simulink model "sm_pump_triplex"  (R2025a)
settings: Solver=VariableStepAuto  StartTime=0.0  StopTime=1.5  RelTol=1e-3  EnableMultiTasking=on
undefined symbols (not defined in the file): pOut_Init_WKSP, smiData, TRP_Par, X, Y, Z
libraries: sm_lib x43, fl_lib x30, nesl_utility x11, simulink x10, SimscapeFluids_lib x3, sm_pump_triplex_lib x3, ee_lib x2, Multibody_Multiphysics_Lib x1
(part 3 of 3)

== system sm_pump_triplex/Pump/Crank/Crankpin 1 ==
  Shaft : sm_lib/Body Elements/Cylindrical Solid  CylinderRadius=shaft_rad  CylinderRadiusUnits=m  CylinderLength=shaft_len  CylinderLengthUnits=m  ExportEntireGeometry=off  InertiaType=CalculateFromGeometry  BasedOnType=Density  Density=crank_rho  DensityUnits=kg/m^3  Mass=1  MassUnits=kg  CenterOfMass=[0 0 0]  CenterOfMassUnits=m  MomentsOfInertia=[1 1 1]  MomentsOfInertiaUnits=kg*m^2  ProductsOfInertia=[1 1 1]  ProductsOfInertiaUnits=kg*m^2  GraphicType=FromGeometry  MarkerShape=Sphere  MarkerSize=10  GraphicVisPropType=SimpleVisualProperties  GraphicDiffuseColor=crank_clr  GraphicOpacity=crank_opc  GraphicSpecularColor=[0.5 0.5 0.5 1.0]  GraphicAmbientColor=[0.15 0.15 0.15 1.0]  GraphicEmissiveColor=[0.0 0.0 0.0 1.0]  GraphicShininess=75  DoExposeReferenceFrame=on  SerializedFrames=<Frames/>
  Transform S1 End : sm_lib/Frames and Transforms/Rigid Transform  RotationMethod=None  FollAlignAxisA=+X  BaseAlignAxisA=+Y  FollAlignAxisB=+Y  BaseAlignAxisB=+Z  RotationStandardAxis=+Z  RotationAngle=0.0  RotationAngleUnits=deg  RotationArbitraryAxis=[0 0 1]  RotationSequenceAxes=FollowerAxes  RotationSequence=XYX  RotationSequenceAngles=[0 0 0]  RotationSequenceAnglesUnits=deg  RotationMatrix=[1 0 0; 0 1 0; 0 0 1]  Quaternion=[1 0 0 0]  TranslationMethod=StandardAxis  TranslationCartesianOffset=[0 0 0]  TranslationCartesianOffsetUnits=m  TranslationStandardAxis=+Z  TranslationStandardOffset=shaft_len/2  TranslationStandardOffsetUnits=m  TranslationROffset=0  TranslationROffsetUnits=m  TranslationThetaOffset=0  TranslationThetaOffsetUnits=deg  TranslationZOffset=0  TranslationZOffsetUnits=m
  Transform S1 End1 : sm_lib/Frames and Transforms/Rigid Transform  RotationMethod=None  FollAlignAxisA=+X  BaseAlignAxisA=+Y  FollAlignAxisB=+Y  BaseAlignAxisB=+Z  RotationStandardAxis=+Z  RotationAngle=0.0  RotationAngleUnits=deg  RotationArbitraryAxis=[0 0 1]  RotationSequenceAxes=FollowerAxes  RotationSequence=XYX  RotationSequenceAngles=[0 0 0]  RotationSequenceAnglesUnits=deg  RotationMatrix=[1 0 0; 0 1 0; 0 0 1]  Quaternion=[1 0 0 0]  TranslationMethod=StandardAxis  TranslationCartesianOffset=[0 0 0]  TranslationCartesianOffsetUnits=m  TranslationStandardAxis=+Z  TranslationStandardOffset=shaft_len/2  TranslationStandardOffsetUnits=m  TranslationROffset=0  TranslationROffsetUnits=m  TranslationThetaOffset=0  TranslationThetaOffsetUnits=deg  TranslationZOffset=0  TranslationZOffsetUnits=m
  Transform Web 1 : sm_lib/Frames and Transforms/Rigid Transform  RotationMethod=None  FollAlignAxisA=+X  BaseAlignAxisA=+Y  FollAlignAxisB=+Y  BaseAlignAxisB=+Z  RotationStandardAxis=+Z  RotationAngle=0.0  RotationAngleUnits=deg  RotationArbitraryAxis=[0 0 1]  RotationSequenceAxes=FollowerAxes  RotationSequence=XYX  RotationSequenceAngles=[0 0 0]  RotationSequenceAnglesUnits=deg  RotationMatrix=[1 0 0; 0 1 0; 0 0 1]  Quaternion=[1 0 0 0]  TranslationMethod=Cylindrical  TranslationCartesianOffset=[0 0 0]  TranslationCartesianOffsetUnits=m  TranslationStandardAxis=+Z  TranslationStandardOffset=0  TranslationStandardOffsetUnits=m  TranslationROffset=shaft_pos  TranslationROffsetUnits=m  TranslationThetaOffset=120  TranslationThetaOffsetUnits=deg  TranslationZOffset=0  TranslationZOffsetUnits=m
  Transform Web 2 : sm_lib/Frames and Transforms/Rigid Transform  RotationMethod=None  FollAlignAxisA=+X  BaseAlignAxisA=+Y  FollAlignAxisB=+Y  BaseAlignAxisB=+Z  RotationStandardAxis=+Z  RotationAngle=0.0  RotationAngleUnits=deg  RotationArbitraryAxis=[0 0 1]  RotationSequenceAxes=FollowerAxes  RotationSequence=XYX  RotationSequenceAngles=[0 0 0]  RotationSequenceAnglesUnits=deg  RotationMatrix=[1 0 0; 0 1 0; 0 0 1]  Quaternion=[1 0 0 0]  TranslationMethod=Cylindrical  TranslationCartesianOffset=[0 0 0]  TranslationCartesianOffsetUnits=m  TranslationStandardAxis=+Z  TranslationStandardOffset=0  TranslationStandardOffsetUnits=m  TranslationROffset=shaft_pos  TranslationROffsetUnits=m  TranslationThetaOffset=-180+120  TranslationThetaOffsetUnits=deg  TranslationZOffset=0  TranslationZOffsetUnits=m
  W2 : PMIOPort  Side=Left
  P1 : PMIOPort  Port=2  Side=Right
  W1 : PMIOPort  Port=3  Side=Left
  connections:
  Transform Web 2/LConn1 -- Transform S1 End1/LConn1
  W2/RConn1 -- Transform Web 2/RConn1
  W1/RConn1 -- Transform Web 1/LConn1
  P1/RConn1 -- Shaft/RConn1 -- Transform S1 End/LConn1 -- Transform S1 End1/RConn1
  Transform Web 1/RConn1 -- Transform S1 End/RConn1

== system sm_pump_triplex/Pump/Crank/Crankpin 2 ==
  Shaft : sm_lib/Body Elements/Cylindrical Solid  CylinderRadius=shaft_rad  CylinderRadiusUnits=m  CylinderLength=shaft_len  CylinderLengthUnits=m  ExportEntireGeometry=off  InertiaType=CalculateFromGeometry  BasedOnType=Density  Density=crank_rho  DensityUnits=kg/m^3  Mass=1  MassUnits=kg  CenterOfMass=[0 0 0]  CenterOfMassUnits=m  MomentsOfInertia=[1 1 1]  MomentsOfInertiaUnits=kg*m^2  ProductsOfInertia=[1 1 1]  ProductsOfInertiaUnits=kg*m^2  GraphicType=FromGeometry  MarkerShape=Sphere  MarkerSize=10  GraphicVisPropType=SimpleVisualProperties  GraphicDiffuseColor=crank_clr  GraphicOpacity=crank_opc  GraphicSpecularColor=[0.5 0.5 0.5 1.0]  GraphicAmbientColor=[0.15 0.15 0.15 1.0]  GraphicEmissiveColor=[0.0 0.0 0.0 1.0]  GraphicShininess=75  DoExposeReferenceFrame=on  SerializedFrames=<Frames/>
  Transform S1 End : sm_lib/Frames and Transforms/Rigid Transform  RotationMethod=None  FollAlignAxisA=+X  BaseAlignAxisA=+Y  FollAlignAxisB=+Y  BaseAlignAxisB=+Z  RotationStandardAxis=+Z  RotationAngle=0.0  RotationAngleUnits=deg  RotationArbitraryAxis=[0 0 1]  RotationSequenceAxes=FollowerAxes  RotationSequence=XYX  RotationSequenceAngles=[0 0 0]  RotationSequenceAnglesUnits=deg  RotationMatrix=[1 0 0; 0 1 0; 0 0 1]  Quaternion=[1 0 0 0]  TranslationMethod=StandardAxis  TranslationCartesianOffset=[0 0 0]  TranslationCartesianOffsetUnits=m  TranslationStandardAxis=+Z  TranslationStandardOffset=shaft_len/2  TranslationStandardOffsetUnits=m  TranslationROffset=0  TranslationROffsetUnits=m  TranslationThetaOffset=0  TranslationThetaOffsetUnits=deg  TranslationZOffset=0  TranslationZOffsetUnits=m
  Transform S1 End1 : sm_lib/Frames and Transforms/Rigid Transform  RotationMethod=None  FollAlignAxisA=+X  BaseAlignAxisA=+Y  FollAlignAxisB=+Y  BaseAlignAxisB=+Z  RotationStandardAxis=+Z  RotationAngle=0.0  RotationAngleUnits=deg  RotationArbitraryAxis=[0 0 1]  RotationSequenceAxes=FollowerAxes  RotationSequence=XYX  RotationSequenceAngles=[0 0 0]  RotationSequenceAnglesUnits=deg  RotationMatrix=[1 0 0; 0 1 0; 0 0 1]  Quaternion=[1 0 0 0]  TranslationMethod=StandardAxis  TranslationCartesianOffset=[0 0 0]  TranslationCartesianOffsetUnits=m  TranslationStandardAxis=+Z  TranslationStandardOffset=shaft_len/2  TranslationStandardOffsetUnits=m  TranslationROffset=0  TranslationROffsetUnits=m  TranslationThetaOffset=0  TranslationThetaOffsetUnits=deg  TranslationZOffset=0  TranslationZOffsetUnits=m
  Transform Web 1 : sm_lib/Frames and Transforms/Rigid Transform  RotationMethod=None  FollAlignAxisA=+X  BaseAlignAxisA=+Y  FollAlignAxisB=+Y  BaseAlignAxisB=+Z  RotationStandardAxis=+Z  RotationAngle=0.0  RotationAngleUnits=deg  RotationArbitraryAxis=[0 0 1]  RotationSequenceAxes=FollowerAxes  RotationSequence=XYX  RotationSequenceAngles=[0 0 0]  RotationSequenceAnglesUnits=deg  RotationMatrix=[1 0 0; 0 1 0; 0 0 1]  Quaternion=[1 0 0 0]  TranslationMethod=Cylindrical  TranslationCartesianOffset=[0 0 0]  TranslationCartesianOffsetUnits=m  TranslationStandardAxis=+Z  TranslationStandardOffset=0  TranslationStandardOffsetUnits=m  TranslationROffset=shaft_pos  TranslationROffsetUnits=m  TranslationThetaOffset=0  TranslationThetaOffsetUnits=deg  TranslationZOffset=0  TranslationZOffsetUnits=m
  Transform Web 2 : sm_lib/Frames and Transforms/Rigid Transform  RotationMethod=None  FollAlignAxisA=+X  BaseAlignAxisA=+Y  FollAlignAxisB=+Y  BaseAlignAxisB=+Z  RotationStandardAxis=+Z  RotationAngle=0.0  RotationAngleUnits=deg  RotationArbitraryAxis=[0 0 1]  RotationSequenceAxes=FollowerAxes  RotationSequence=XYX  RotationSequenceAngles=[0 0 0]  RotationSequenceAnglesUnits=deg  RotationMatrix=[1 0 0; 0 1 0; 0 0 1]  Quaternion=[1 0 0 0]  TranslationMethod=Cylindrical  TranslationCartesianOffset=[0 0 0]  TranslationCartesianOffsetUnits=m  TranslationStandardAxis=+Z  TranslationStandardOffset=0  TranslationStandardOffsetUnits=m  TranslationROffset=shaft_pos  TranslationROffsetUnits=m  TranslationThetaOffset=-180  TranslationThetaOffsetUnits=deg  TranslationZOffset=0  TranslationZOffsetUnits=m
  W2 : PMIOPort  Side=Left
  P1 : PMIOPort  Port=2  Side=Right
  W1 : PMIOPort  Port=3  Side=Left
  connections:
  Transform Web 1/RConn1 -- Transform S1 End/RConn1
  Transform S1 End1/RConn1 -- Transform S1 End/LConn1 -- Shaft/RConn1 -- P1/RConn1
  W1/RConn1 -- Transform Web 1/LConn1
  W2/RConn1 -- Transform Web 2/RConn1
  Transform Web 2/LConn1 -- Transform S1 End1/LConn1

== system sm_pump_triplex/Pump/Crank/Crankpin 3 ==
  Shaft : sm_lib/Body Elements/Cylindrical Solid  CylinderRadius=shaft_rad  CylinderRadiusUnits=m  CylinderLength=shaft_len  CylinderLengthUnits=m  ExportEntireGeometry=off  InertiaType=CalculateFromGeometry  BasedOnType=Density  Density=crank_rho  DensityUnits=kg/m^3  Mass=1  MassUnits=kg  CenterOfMass=[0 0 0]  CenterOfMassUnits=m  MomentsOfInertia=[1 1 1]  MomentsOfInertiaUnits=kg*m^2  ProductsOfInertia=[1 1 1]  ProductsOfInertiaUnits=kg*m^2  GraphicType=FromGeometry  MarkerShape=Sphere  MarkerSize=10  GraphicVisPropType=SimpleVisualProperties  GraphicDiffuseColor=crank_clr  GraphicOpacity=crank_opc  GraphicSpecularColor=[0.5 0.5 0.5 1.0]  GraphicAmbientColor=[0.15 0.15 0.15 1.0]  GraphicEmissiveColor=[0.0 0.0 0.0 1.0]  GraphicShininess=75  DoExposeReferenceFrame=on  SerializedFrames=<Frames/>
  Transform S1 End : sm_lib/Frames and Transforms/Rigid Transform  RotationMethod=None  FollAlignAxisA=+X  BaseAlignAxisA=+Y  FollAlignAxisB=+Y  BaseAlignAxisB=+Z  RotationStandardAxis=+Z  RotationAngle=0.0  RotationAngleUnits=deg  RotationArbitraryAxis=[0 0 1]  RotationSequenceAxes=FollowerAxes  RotationSequence=XYX  RotationSequenceAngles=[0 0 0]  RotationSequenceAnglesUnits=deg  RotationMatrix=[1 0 0; 0 1 0; 0 0 1]  Quaternion=[1 0 0 0]  TranslationMethod=StandardAxis  TranslationCartesianOffset=[0 0 0]  TranslationCartesianOffsetUnits=m  TranslationStandardAxis=+Z  TranslationStandardOffset=shaft_len/2  TranslationStandardOffsetUnits=m  TranslationROffset=0  TranslationROffsetUnits=m  TranslationThetaOffset=0  TranslationThetaOffsetUnits=deg  TranslationZOffset=0  TranslationZOffsetUnits=m
  Transform S1 End1 : sm_lib/Frames and Transforms/Rigid Transform  RotationMethod=None  FollAlignAxisA=+X  BaseAlignAxisA=+Y  FollAlignAxisB=+Y  BaseAlignAxisB=+Z  RotationStandardAxis=+Z  RotationAngle=0.0  RotationAngleUnits=deg  RotationArbitraryAxis=[0 0 1]  RotationSequenceAxes=FollowerAxes  RotationSequence=XYX  RotationSequenceAngles=[0 0 0]  RotationSequenceAnglesUnits=deg  RotationMatrix=[1 0 0; 0 1 0; 0 0 1]  Quaternion=[1 0 0 0]  TranslationMethod=StandardAxis  TranslationCartesianOffset=[0 0 0]  TranslationCartesianOffsetUnits=m  TranslationStandardAxis=+Z  TranslationStandardOffset=shaft_len/2  TranslationStandardOffsetUnits=m  TranslationROffset=0  TranslationROffsetUnits=m  TranslationThetaOffset=0  TranslationThetaOffsetUnits=deg  TranslationZOffset=0  TranslationZOffsetUnits=m
  Transform Web 1 : sm_lib/Frames and Transforms/Rigid Transform  RotationMethod=None  FollAlignAxisA=+X  BaseAlignAxisA=+Y  FollAlignAxisB=+Y  BaseAlignAxisB=+Z  RotationStandardAxis=+Z  RotationAngle=0.0  RotationAngleUnits=deg  RotationArbitraryAxis=[0 0 1]  RotationSequenceAxes=FollowerAxes  RotationSequence=XYX  RotationSequenceAngles=[0 0 0]  RotationSequenceAnglesUnits=deg  RotationMatrix=[1 0 0; 0 1 0; 0 0 1]  Quaternion=[1 0 0 0]  TranslationMethod=Cylindrical  TranslationCartesianOffset=[0 0 0]  TranslationCartesianOffsetUnits=m  TranslationStandardAxis=+Z  TranslationStandardOffset=0  TranslationStandardOffsetUnits=m  TranslationROffset=shaft_pos  TranslationROffsetUnits=m  TranslationThetaOffset=-120  TranslationThetaOffsetUnits=deg  TranslationZOffset=0  TranslationZOffsetUnits=m
  Transform Web 2 : sm_lib/Frames and Transforms/Rigid Transform  RotationMethod=None  FollAlignAxisA=+X  BaseAlignAxisA=+Y  FollAlignAxisB=+Y  BaseAlignAxisB=+Z  RotationStandardAxis=+Z  RotationAngle=0.0  RotationAngleUnits=deg  RotationArbitraryAxis=[0 0 1]  RotationSequenceAxes=FollowerAxes  RotationSequence=XYX  RotationSequenceAngles=[0 0 0]  RotationSequenceAnglesUnits=deg  RotationMatrix=[1 0 0; 0 1 0; 0 0 1]  Quaternion=[1 0 0 0]  TranslationMethod=Cylindrical  TranslationCartesianOffset=[0 0 0]  TranslationCartesianOffsetUnits=m  TranslationStandardAxis=+Z  TranslationStandardOffset=0  TranslationStandardOffsetUnits=m  TranslationROffset=shaft_pos  TranslationROffsetUnits=m  TranslationThetaOffset=-180-120  TranslationThetaOffsetUnits=deg  TranslationZOffset=0  TranslationZOffsetUnits=m
  W2 : PMIOPort  Side=Left
  P1 : PMIOPort  Port=2  Side=Right
  W1 : PMIOPort  Port=3  Side=Left
  connections:
  Transform Web 2/LConn1 -- Transform S1 End1/LConn1
  W2/RConn1 -- Transform Web 2/RConn1
  W1/RConn1 -- Transform Web 1/LConn1
  P1/RConn1 -- Shaft/RConn1 -- Transform S1 End/LConn1 -- Transform S1 End1/RConn1
  Transform Web 1/RConn1 -- Transform S1 End/RConn1

== system sm_pump_triplex/Pump/Housing/Bearing Fault Visual ==
  Bearing Fault Visual L : sm_lib/Body Elements/Cylindrical Solid  CylinderRadius=bearing_fault_vis_rad  CylinderRadiusUnits=m  CylinderLength=bearing_fault_vis_len  CylinderLengthUnits=m  ExportEntireGeometry=off  InertiaType=CalculateFromGeometry  BasedOnType=Density  Density=0.001  DensityUnits=kg/m^3  Mass=1  MassUnits=kg  CenterOfMass=[0 0 0]  CenterOfMassUnits=m  MomentsOfInertia=[1 1 1]  MomentsOfInertiaUnits=kg*m^2  ProductsOfInertia=[1 1 1]  ProductsOfInertiaUnits=kg*m^2  GraphicType=FromGeometry  MarkerShape=Sphere  MarkerSize=10  GraphicVisPropType=SimpleVisualProperties  GraphicDiffuseColor=bearing_fault_vis_clr  GraphicOpacity=bearing_fault_vis_opc  GraphicSpecularColor=[0.5 0.5 0.5 1.0]  GraphicAmbientColor=[0.15 0.15 0.15 1.0]  GraphicEmissiveColor=[0.0 0.0 0.0 1.0]  GraphicShininess=75  DoExposeReferenceFrame=on  SerializedFrames=<Frames/>
  Bearing Fault Visual R : sm_lib/Body Elements/Cylindrical Solid  CylinderRadius=bearing_fault_vis_rad  CylinderRadiusUnits=m  CylinderLength=bearing_fault_vis_len  CylinderLengthUnits=m  ExportEntireGeometry=off  InertiaType=CalculateFromGeometry  BasedOnType=Density  Density=0.001  DensityUnits=kg/m^3  Mass=1  MassUnits=kg  CenterOfMass=[0 0 0]  CenterOfMassUnits=m  MomentsOfInertia=[1 1 1]  MomentsOfInertiaUnits=kg*m^2  ProductsOfInertia=[1 1 1]  ProductsOfInertiaUnits=kg*m^2  GraphicType=FromGeometry  MarkerShape=Sphere  MarkerSize=10  GraphicVisPropType=SimpleVisualProperties  GraphicDiffuseColor=bearing_fault_vis_clr  GraphicOpacity=bearing_fault_vis_opc  GraphicSpecularColor=[0.5 0.5 0.5 1.0]  GraphicAmbientColor=[0.15 0.15 0.15 1.0]  GraphicEmissiveColor=[0.0 0.0 0.0 1.0]  GraphicShininess=75  DoExposeReferenceFrame=on  SerializedFrames=<Frames/>
  Transform Bearing Fault L : sm_lib/Frames and Transforms/Rigid Transform  RotationMethod=None  FollAlignAxisA=+X  BaseAlignAxisA=+Y  FollAlignAxisB=+Y  BaseAlignAxisB=+Z  RotationStandardAxis=+Z  RotationAngle=0.0  RotationAngleUnits=deg  RotationArbitraryAxis=[0 0 1]  RotationSequenceAxes=FollowerAxes  RotationSequence=XYX  RotationSequenceAngles=[0 0 0]  RotationSequenceAnglesUnits=deg  RotationMatrix=[1 0 0; 0 1 0; 0 0 1]  Quaternion=[1 0 0 0]  TranslationMethod=StandardAxis  TranslationCartesianOffset=[0 0 0]  TranslationCartesianOffsetUnits=m  TranslationStandardAxis=+Z  TranslationStandardOffset=bearing_sep/2  TranslationStandardOffsetUnits=m  TranslationROffset=0  TranslationROffsetUnits=m  TranslationThetaOffset=0  TranslationThetaOffsetUnits=deg  TranslationZOffset=0  TranslationZOffsetUnits=m
  Transform Bearing Fault R : sm_lib/Frames and Transforms/Rigid Transform  RotationMethod=None  FollAlignAxisA=+X  BaseAlignAxisA=+Y  FollAlignAxisB=+Y  BaseAlignAxisB=+Z  RotationStandardAxis=+Z  RotationAngle=0.0  RotationAngleUnits=deg  RotationArbitraryAxis=[0 0 1]  RotationSequenceAxes=FollowerAxes  RotationSequence=XYX  RotationSequenceAngles=[0 0 0]  RotationSequenceAnglesUnits=deg  RotationMatrix=[1 0 0; 0 1 0; 0 0 1]  Quaternion=[1 0 0 0]  TranslationMethod=StandardAxis  TranslationCartesianOffset=[0 0 0]  TranslationCartesianOffsetUnits=m  TranslationStandardAxis=-Z  TranslationStandardOffset=bearing_sep/2  TranslationStandardOffsetUnits=m  TranslationROffset=0  TranslationROffsetUnits=m  TranslationThetaOffset=0  TranslationThetaOffsetUnits=deg  TranslationZOffset=0  TranslationZOffsetUnits=m
  C : PMIOPort  Side=Left
  connections:
  Transform Bearing Fault L/LConn1 -- Transform Bearing Fault R/LConn1 -- C/RConn1
  Bearing Fault Visual R/RConn1 -- Transform Bearing Fault R/RConn1
  Bearing Fault Visual L/RConn1 -- Transform Bearing Fault L/RConn1

== system sm_pump_triplex/Pump/Housing/Shell ==
  Housing_1_RIGID : Subsystem
  Manifold_1_RIGID : Subsystem
  Transform : sm_lib/Frames and Transforms/Rigid Transform  RotationMethod=ArbitraryAxis  FollAlignAxisA=+X  BaseAlignAxisA=+Y  FollAlignAxisB=+Y  BaseAlignAxisB=+Z  RotationStandardAxis=+Z  RotationAngle=smiData.RigidTransform(9).angle  RotationAngleUnits=rad  RotationArbitraryAxis=smiData.RigidTransform(9).axis  RotationSequenceAxes=FollowerAxes  RotationSequence=XYX  RotationSequenceAngles=[0 0 0]  RotationSequenceAnglesUnits=deg  RotationMatrix=[1 0 0; 0 1 0; 0 0 1]  Quaternion=[1 0 0 0]  TranslationMethod=Cartesian  TranslationCartesianOffset=smiData.RigidTransform(9).translation  TranslationCartesianOffsetUnits=in  TranslationStandardAxis=+Z  TranslationStandardOffset=0  TranslationStandardOffsetUnits=in  TranslationROffset=0  TranslationROffsetUnits=m  TranslationThetaOffset=0  TranslationThetaOffsetUnits=deg  TranslationZOffset=0  TranslationZOffsetUnits=m
  Transform1 : sm_lib/Frames and Transforms/Rigid Transform  RotationMethod=ArbitraryAxis  FollAlignAxisA=+X  BaseAlignAxisA=+Y  FollAlignAxisB=+Y  BaseAlignAxisB=+Z  RotationStandardAxis=+Z  RotationAngle=smiData.RigidTransform(10).angle  RotationAngleUnits=rad  RotationArbitraryAxis=smiData.RigidTransform(10).axis  RotationSequenceAxes=FollowerAxes  RotationSequence=XYX  RotationSequenceAngles=[0 0 0]  RotationSequenceAnglesUnits=deg  RotationMatrix=[1 0 0; 0 1 0; 0 0 1]  Quaternion=[1 0 0 0]  TranslationMethod=Cartesian  TranslationCartesianOffset=smiData.RigidTransform(10).translation  TranslationCartesianOffsetUnits=in  TranslationStandardAxis=+Z  TranslationStandardOffset=0  TranslationStandardOffsetUnits=in  TranslationROffset=0  TranslationROffsetUnits=m  TranslationThetaOffset=0  TranslationThetaOffsetUnits=deg  TranslationZOffset=0  TranslationZOffsetUnits=m
  W : PMIOPort  Side=Left
  connections:
  Transform1/LConn1 -- W/RConn1 -- Transform/LConn1
  Manifold_1_RIGID/LConn1 -- Transform/RConn1
  Housing_1_RIGID/LConn1 -- Transform1/RConn1

== system sm_pump_triplex/Driver/Driver/Dyno/Sensing Speed ==
  w : Inport
  Measurement Noise : simulink/Sources/Band-Limited White Noise  Cov=TRP_Par.Sensors.w.Np  Ts=TRP_Par.Sensors.w.Ts  seed=[23345]
  Motor Gear Ratio : Gain  Gain=TRP_Par.Motor.Gear.ratio
  Speed with Noise : Scope  NumInputPorts=2
      settings: ActiveDisplayYMinimum=-126.98875  ActiveDisplayYMaximum=1142.56233
  Sum1 : Sum  Inputs=++|
  Zero-Order Hold : ZeroOrderHold  SampleTime=TRP_Par.Sensors.w.Ts
  wires:
  Measurement Noise/1 -> Sum1/1  "Noise"
  w/1 -> Motor Gear Ratio/1
  Sum1/1 -> Zero-Order Hold/1
  Zero-Order Hold/1 -> Speed with Noise/1
  Motor Gear Ratio/1 -> Sum1/2, Speed with Noise/2

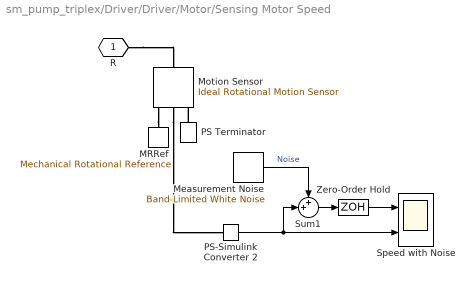
== system sm_pump_triplex/Driver/Driver/Motor/Sensing Motor Speed ==
  MRRef : fl_lib/Mechanical/Rotational Elements/Mechanical Rotational Reference
  Measurement Noise : simulink/Sources/Band-Limited White Noise  Cov=TRP_Par.Sensors.w.Np  Ts=TRP_Par.Sensors.w.Ts  seed=[23345]
  Motion Sensor : fl_lib/Mechanical/Mechanical Sensors/Ideal Rotational Motion Sensor  reference=foundation.enum.MeasurementReference.difference  acceleration_port=false  velocity_port=true  position_port=true  wrap_angle=simscape.enum.onoff.off  offset=0 rad
  PS Terminator : fl_lib/Physical Signals/Sinks/PS Terminator
  PS-Simulink Converter 2 : nesl_utility/PS-Simulink Converter  PhysicalDomain=network_engine_domain  SubClassName=ps_output  LeftPortType=input  RightPortType=output  PseudoPeriodic=off  Frequencies=[]  VectorFormat=1-D array  Unit=rpm  AffineConversion=off
  Speed with Noise : Scope  NumInputPorts=2
      settings: ActiveDisplayYMinimum=-126.98875  ActiveDisplayYMaximum=1142.56233
  Sum1 : Sum  Inputs=++|
  Zero-Order Hold : ZeroOrderHold  SampleTime=TRP_Par.Sensors.w.Ts
  R : PMIOPort  Side=Left
  wires:
  Measurement Noise/1 -> Sum1/1  "Noise"
  PS-Simulink Converter 2/1 -> Speed with Noise/2, Sum1/2
  Zero-Order Hold/1 -> Speed with Noise/1
  Sum1/1 -> Zero-Order Hold/1
  connections:
  PS Terminator/LConn1 -- Motion Sensor/RConn3
  R/RConn1 -- Motion Sensor/LConn1
  Motion Sensor/RConn1 -- MRRef/LConn1
  Motion Sensor/RConn2 -- PS-Simulink Converter 2/LConn1

== system sm_pump_triplex/Driver/Driver/Motor/Sensing Pump Speed ==
  MRRef : fl_lib/Mechanical/Rotational Elements/Mechanical Rotational Reference
  Motion Sensor : fl_lib/Mechanical/Mechanical Sensors/Ideal Rotational Motion Sensor  reference=foundation.enum.MeasurementReference.difference  acceleration_port=false  velocity_port=true  position_port=true  wrap_angle=simscape.enum.onoff.off  offset=0 rad
  PS-Simulink Converter 1 : nesl_utility/PS-Simulink Converter  PhysicalDomain=network_engine_domain  SubClassName=ps_output  LeftPortType=input  RightPortType=output  PseudoPeriodic=off  Frequencies=[]  VectorFormat=1-D array  Unit=deg  AffineConversion=off
  PS-Simulink Converter 2 : nesl_utility/PS-Simulink Converter  PhysicalDomain=network_engine_domain  SubClassName=ps_output  LeftPortType=input  RightPortType=output  PseudoPeriodic=off  Frequencies=[]  VectorFormat=1-D array  Unit=rpm  AffineConversion=off
  R : PMIOPort  Side=Left
  A : Outport  VectorParamsAs1DForOutWhenUnconnected=off
  rpm : Outport  Port=2  VectorParamsAs1DForOutWhenUnconnected=off
  wires:
  PS-Simulink Converter 1/1 -> A/1
  PS-Simulink Converter 2/1 -> rpm/1
  connections:
  Motion Sensor/RConn2 -- PS-Simulink Converter 2/LConn1
  Motion Sensor/RConn1 -- MRRef/LConn1
  R/RConn1 -- Motion Sensor/LConn1
  Motion Sensor/RConn3 -- PS-Simulink Converter 1/LConn1

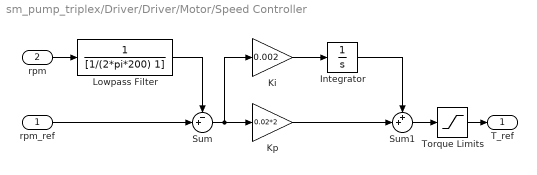
== system sm_pump_triplex/Driver/Driver/Motor/Speed Controller ==
  rpm_ref : Inport
  rpm : Inport  Port=2
  Integrator : Integrator  LimitOutput=on  UpperSaturationLimit=40  LowerSaturationLimit=-40
      settings: AttributesFormatString=Saturate: [%<LowerSaturationLimit>, %<UpperSaturationLimit>]
  Ki : Gain  Gain=0.002
  Kp : Gain  Gain=0.02*2
  Lowpass Filter : TransferFcn  Denominator=[1/(2*pi*200) 1]
  Sum : Sum  Inputs=-+|
  Sum1 : Sum  Inputs=++|
  Torque Limits : Saturate  UpperLimit=400  LowerLimit=-400
  T_ref : Outport  VectorParamsAs1DForOutWhenUnconnected=off
  wires:
  rpm_ref/1 -> Sum/2
  rpm/1 -> Lowpass Filter/1
  Sum1/1 -> Torque Limits/1
  Sum/1 -> Ki/1, Kp/1
  Ki/1 -> Integrator/1
  Kp/1 -> Sum1/2
  Integrator/1 -> Sum1/1
  Lowpass Filter/1 -> Sum/1
  Torque Limits/1 -> T_ref/1

== system sm_pump_triplex/Driver/Driver/Motor/Windings ==
  T_ref : Inport
  deg : Inport  Port=2
  Constant : Constant  Value=winding_fault_sw
  Constant1 : Constant
  Enable if rotor angle 0-240 Deg : Subsystem
  Product : Product
  Switch : Switch  Criteria=u2 > Threshold  Threshold=1.5  SaturateOnIntegerOverflow=off  InputSameDT=off
  Unit Delay : UnitDelay  SampleTime=0.001  HasFrameUpgradeWarning=on
  Trq : Outport  VectorParamsAs1DForOutWhenUnconnected=off
  wires:
  Product/1 -> Trq/1
  T_ref/1 -> Product/1
  Constant/1 -> Switch/2
  Constant1/1 -> Switch/3
  Switch/1 -> Product/2
  deg/1 -> Unit Delay/1
  Enable if rotor angle 0-240 Deg/1(En) -> Switch/1
  Unit Delay/1 -> Enable if rotor angle 0-240 Deg/1(Ang)

== system sm_pump_triplex/Pump/Housing/Shell/Housing_1_RIGID ==
  ReferenceFrame : sm_lib/Frames and Transforms/Reference Frame
  Solid : sm_lib/Body Elements/File Solid  ExtGeomFileName=Housing_Default_sldprt.STEP  UnitType=FromFile  ExtGeomFileUnits=m  StepReaderType=HEX  ExportConvexHullGeometry=off  InertiaType=Custom  BasedOnType=Density  Density=1000  DensityUnits=kg/m^3  Mass=smiData.Solid(4).mass  MassUnits=kg  CenterOfMass=smiData.Solid(4).CoM  CenterOfMassUnits=in  MomentsOfInertia=smiData.Solid(4).MoI  MomentsOfInertiaUnits=kg*in^2  ProductsOfInertia=smiData.Solid(4).PoI  ProductsOfInertiaUnits=kg*in^2  GraphicType=FromGeometry  MarkerShape=Sphere  MarkerSize=10  GraphicVisPropType=SimpleVisualProperties  GraphicDiffuseColor=housing_clr  GraphicOpacity=housing_opc  GraphicSpecularColor=[0.5 0.5 0.5 1.0]  GraphicAmbientColor=[0.15 0.15 0.15 1.0]  GraphicEmissiveColor=[0.0 0.0 0.0 1.0]  GraphicShininess=75  DoExposeReferenceFrame=on  SerializedFrames=<Frames/>
  F : PMIOPort  Side=Left
  connections:
  Solid/RConn1 -- ReferenceFrame/RConn1 -- F/RConn1

== system sm_pump_triplex/Pump/Housing/Shell/Manifold_1_RIGID ==
  ReferenceFrame : sm_lib/Frames and Transforms/Reference Frame
  Solid : sm_lib/Body Elements/File Solid  ExtGeomFileName=Manifold_Default_sldprt.STEP  UnitType=FromFile  ExtGeomFileUnits=m  StepReaderType=HEX  ExportConvexHullGeometry=off  InertiaType=Custom  BasedOnType=Density  Density=1000  DensityUnits=kg/m^3  Mass=smiData.Solid(3).mass  MassUnits=kg  CenterOfMass=smiData.Solid(3).CoM  CenterOfMassUnits=in  MomentsOfInertia=smiData.Solid(3).MoI  MomentsOfInertiaUnits=kg*in^2  ProductsOfInertia=smiData.Solid(3).PoI  ProductsOfInertiaUnits=kg*in^2  GraphicType=FromGeometry  MarkerShape=Sphere  MarkerSize=10  GraphicVisPropType=SimpleVisualProperties  GraphicDiffuseColor=manifold_clr  GraphicOpacity=manifold_opc  GraphicSpecularColor=[0.5 0.5 0.5 1.0]  GraphicAmbientColor=[0.15 0.15 0.15 1.0]  GraphicEmissiveColor=[0.0 0.0 0.0 1.0]  GraphicShininess=75  DoExposeReferenceFrame=on  SerializedFrames=<Frames/>
  F : PMIOPort  Side=Left
  connections:
  Solid/RConn1 -- ReferenceFrame/RConn1 -- F/RConn1

== system sm_pump_triplex/Driver/Driver/Motor/Windings/Enable if rotor angle 0-240 Deg ==
  Ang : Inport
  Constant2 : Constant  Value=360
  Interval Test : simulink/Logic and Bit Operations/Interval Test  IntervalClosedRight=on  uplimit=240  IntervalClosedLeft=on  lowlimit=0  OutDataTypeStr=uint8
      settings: AttributesFormatString=%<lowlimit><angle<%<uplimit>
  Math Function : Math  Operator=rem  SignedPower=on
  En : Outport  VectorParamsAs1DForOutWhenUnconnected=off
  wires:
  Constant2/1 -> Math Function/2
  Math Function/1 -> Interval Test/1
  Interval Test/1 -> En/1
  Ang/1 -> Math Function/1

== matlab function sm_pump_triplex/Diagnostics/Diagnostics/On/FFT and Classification ==
  data: pArray input; faultState output; enablePred input; cmdSpeed input; hmiVec output
function [faultState,hmiVec] = faultClassifier(pArray,enablePred,cmdSpeed)

% Initialize Predicted Machine State
faultState = int8(0);
hmiVec = [1 0 0 0];

% Sampling Parameters
Np = 1000;
Dt = 0.001;
numFreqPeaks = 5;

% Initialize Prediction Algorithm Input
predIn = NaN(1,2*numFreqPeaks+1);

pAvg = mean(pArray);

% Load Trained Machine Learning Algorithm
pumpPredict = loadLearnerForCoder('sm_pump_triplex_fault_detect_algo');

if enablePred
    
    % Compute FFT of Accumulated Data
    [freq,mag] = getFFTData(Np,pArray,Dt);
    
    % Normalize FFT Results
    freqFaultSpd = freq*60/(2*pi)/(cmdSpeed*3);

    % Detect FFT Peak Frequencies
    [pks,loc] = findpeaks(mag,'MinPeakProminence',0.5e-3);

    % Center FFT Peak Frequencies around Primary Machine Frequency
    normSpd = abs(freqFaultSpd(loc)-1);
    [sortFreq,sortIdx] = sort(normSpd);
    sortMag = pks(sortIdx);

    % Only Update Detected Peaks
    if length(sortMag) <= numFreqPeaks
        numFreq = length(sortMag);
    else
        numFreq = numFreqPeaks;
    end
    
    % Construct Input Array for Machine Learning Algorithm
    for i = 1:numFreq
        predIn(2*(i-1)+1) = sortFreq(i);
        predIn(2*i) = sortMag(i);
        predIn(i+1) = sortMag(i);
    end
    predIn(2*numFreqPeaks+1) = pAvg;
    
    % Predict Machine State using Classification Algorithm
    faultState = predict(pumpPredict,predIn);
    
    % Flag Machine Vector for HMI Indicators
    if faultState == 3 || faultState == 4 || faultState == 5
        hmiVec(2) = 1;  hmiVec(1) = 0;
    end
    if faultState == 1 || faultState == 2 || faultState == 4
        hmiVec(3) = 1;  hmiVec(1) = 0;
    end
    if faultState == 2 || faultState == 5 || faultState == 7
        hmiVec(4) = 1;  hmiVec(1) = 0;
    end
    
else
    % 
    faultState = int8(0);
    hmiVec = [0 0 0 0];
end
end

function [freq, mag] = getFFTData(np,yout,dt)
% Code to calculate frequency response data
%
% Copyright 2017 The MathWorks, Inc.

% % Compute fft
yout_intp = yout(:).*hamming(np);
f = fft(yout_intp)/np;
f2 = f(1:(np/2)+1);
w = (0:np/2)/np*(2*pi/dt);
P = abs(f2);
ind = 20 < w & w < 525; % Between 20 & 525 radians/sec
freq = w(ind)';
mag = P(ind);
end

== matlab function sm_pump_triplex/Diagnostics/Diagnostics/On/Collect Data ==
  data: pOut input; pArray output
function pArray  = dataAccum(pOut)

persistent pOutArray

Np = 1000;

if isempty(pOutArray)
    pOutArray = zeros(Np,1);
end

pOutArray = [pOut; pOutArray(1:Np-1)];
pArray = pOutArray;
end
